simulink model "cable_driven_parallel_robot"  (R2023a)
settings: Solver=ode3  StartTime=0.0  StopTime=100  FixedStep=0.01  RelTol=1e-3
values from neighbouring files (symbols this model uses):
  cable_length = 1.2    [Model_Info.m]
  g = 9.81    [Model_Info.m]
  MP_H = 2    [Model_Info.m]
  MP_init_X = 0    [Model_Info.m]
  MP_init_Y = 0    [Model_Info.m]
  MP_init_Z = cable_length + (MP_H/2)    (= 2.2)    [Model_Info.m]
  MP_Ix = (MP_m/12)*(MP_W^2+MP_H^2)    (= 6.66666666667e-05)    [Model_Info.m]
  MP_Iy = (MP_m/12)*(MP_L^2+MP_H^2)    (= 6.66666666667e-05)    [Model_Info.m]
  MP_Iz = (MP_m/12)*(MP_L^2+MP_W^2)    (= 6.66666666667e-05)    [Model_Info.m]
  MP_L = 2    [Model_Info.m]
  MP_m = 0.0001    [Model_Info.m]
  MP_W = 2    [Model_Info.m]
  MR_init_X_L1 = -(MP_L/2)    (= -1)    [Model_Info.m]
  MR_init_X_L2 = (MP_L/2)    (= 1)    [Model_Info.m]
  MR_init_X_L3 = (MP_L/2)    (= 1)    [Model_Info.m]
  MR_init_X_L4 = -(MP_L/2)    (= -1)    [Model_Info.m]
  MR_init_Y_L1 = -(MP_W/2)    (= -1)    [Model_Info.m]
  MR_init_Y_L2 = -(MP_W/2)    (= -1)    [Model_Info.m]
  MR_init_Y_L3 = (MP_W/2)    (= 1)    [Model_Info.m]
  MR_init_Y_L4 = (MP_W/2)    (= 1)    [Model_Info.m]
  MR_init_Yaw_L1 = pi    (= 3.14159265359)    [Model_Info.m]
  MR_init_Yaw_L2 = 0    [Model_Info.m]
  MR_init_Yaw_L3 = 0    [Model_Info.m]
  MR_init_Yaw_L4 = pi    (= 3.14159265359)    [Model_Info.m]
  MR_Jr = (MR_m/12)*(MR_L^2+MR_W^2)    (= 0.333333333333)    [Model_Info.m]
  MR_m = 0.5    [Model_Info.m]
  MR_r = 2    [Model_Info.m]
  MR_WT = 2    [Model_Info.m]
  QR_Ax = 0.25*0    (= 0)    [Model_Info.m]
  QR_Ay = 0.25*0    (= 0)    [Model_Info.m]
  QR_Az = 0.25*0    (= 0)    [Model_Info.m]
  QR_b = 1.14*1e-7    (= 1.14e-07)    [Model_Info.m]
  QR_Ixx = 4.856*1e-3    (= 0.004856)    [Model_Info.m]
  QR_Iyy = 4.856*1e-3    (= 0.004856)    [Model_Info.m]
  QR_Izz = 8.801*1e-3    (= 0.008801)    [Model_Info.m]
  QR_K = 2.980*1e-6    (= 2.98e-06)    [Model_Info.m]
  QR_l = 0.225    [Model_Info.m]
  QR_m = 0.468    [Model_Info.m]
  QR_x0_U1 = -(MP_L/2)    (= -1)    [Model_Info.m]
  QR_x0_U2 = (MP_L/2)    (= 1)    [Model_Info.m]
  QR_x0_U3 = (MP_L/2)    (= 1)    [Model_Info.m]
  QR_x0_U4 = -(MP_L/2)    (= -1)    [Model_Info.m]
  QR_y0_U1 = -(MP_W/2)    (= -1)    [Model_Info.m]
  QR_y0_U2 = -(MP_W/2)    (= -1)    [Model_Info.m]
  QR_y0_U3 = (MP_W/2)    (= 1)    [Model_Info.m]
  QR_y0_U4 = (MP_W/2)    (= 1)    [Model_Info.m]
  QR_z0_U1 = 2*cable_length+(MP_H)    (= 4.4)    [Model_Info.m]
  QR_z0_U2 = 2*cable_length+(MP_H)    (= 4.4)    [Model_Info.m]
  QR_z0_U3 = 2*cable_length+(MP_H)    (= 4.4)    [Model_Info.m]
  QR_z0_U4 = 2*cable_length+(MP_H)    (= 4.4)    [Model_Info.m]
(part 4 of 12)

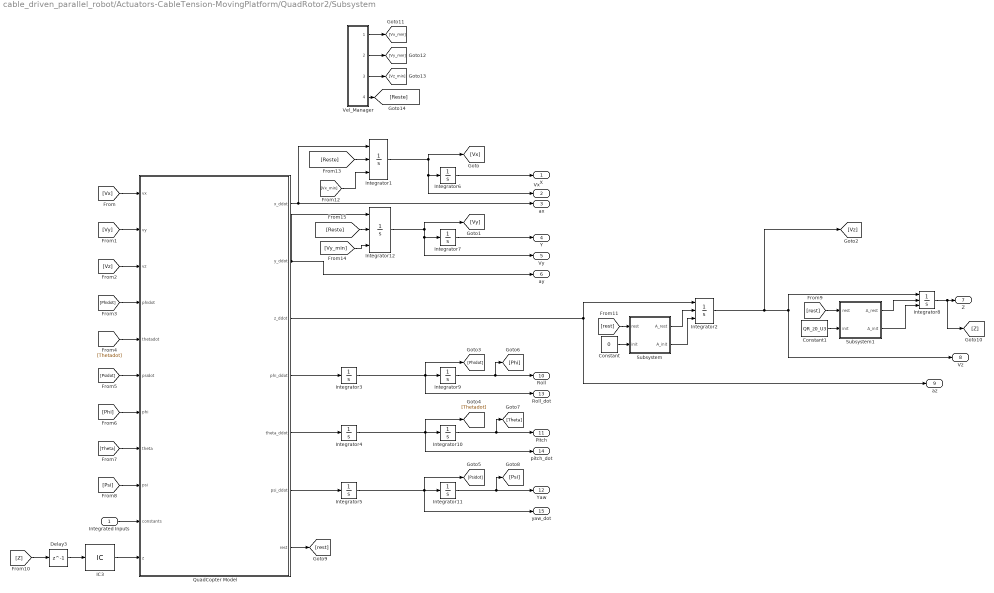
== system cable_driven_parallel_robot/Actuators-CableTension-MovingPlatform/QuadRotor2/Subsystem ==
  Integrated Inputs : Inport
  Constant : Constant  Value=0
  Constant1 : Constant  Value=QR_z0_U3
  Delay3 : Delay  DelayLength=1
  IC3 : InitialCondition  Value=QR_z0_U3
  Integrator1 : Integrator  ExternalReset=rising  InitialConditionSource=external
  Integrator{3..5,9..11} (6 alike) : Integrator
  Integrator12 : Integrator  ExternalReset=rising  InitialConditionSource=external
  Integrator2 : Integrator  ExternalReset=rising  InitialConditionSource=external
  Integrator6 : Integrator  InitialCondition=QR_x0_U3
  Integrator7 : Integrator  InitialCondition=QR_y0_U3
  Integrator8 : Integrator  ExternalReset=rising  InitialConditionSource=external  InitialCondition=QR_z0_U1
  QuadCopter Model : MATLAB Function  TreatAsAtomicUnit=on
  Subsystem : Subsystem
  Subsystem1 : Subsystem
  Vel_Manager : Subsystem
  X : Outport
  Vx : Outport  Port=2
  ax : Outport  Port=3
  Y : Outport  Port=4
  Vy : Outport  Port=5
  ay : Outport  Port=6
  Z : Outport  Port=7
  Vz : Outport  Port=8
  az : Outport  Port=9
  Roll : Outport  Port=10
  Pitch : Outport  Port=11
  Yaw : Outport  Port=12
  Roll_dot : Outport  Port=13
  pitch_dot : Outport  Port=14
  yaw_dot : Outport  Port=15
  wires:
  QuadCopter Model/4(phi_ddot) -> Integrator3/1
  Integrator9/1 -> [Phi], Roll/1
  Integrator4/1 -> pitch_dot/1, [Thetadot], Integrator10/1
  QuadCopter Model/6(psi_ddot) -> Integrator5/1
  Integrator5/1 -> yaw_dot/1, [Psidot], Integrator11/1
  Integrator3/1 -> Roll_dot/1, [Phidot], Integrator9/1
  Integrator1/1 -> [Vx], Vx/1, Integrator6/1
  Integrator10/1 -> [Theta], Pitch/1
  QuadCopter Model/5(theta_ddot) -> Integrator4/1
  QuadCopter Model/2(y_ddot) -> Integrator12/1, ay/1
  QuadCopter Model/1(x_ddot) -> Integrator1/1, ax/1
  Integrator11/1 -> [Psi], Yaw/1
  Integrator6/1 -> X/1
  Integrator7/1 -> Y/1
  Integrator8/1 -> [Z], Z/1
  Integrated Inputs/1 -> QuadCopter Model/10(constants)
  [Vx] -> QuadCopter Model/1(vx)
  [Vy] -> QuadCopter Model/2(vy)
  [Vz] -> QuadCopter Model/3(vz)
  [Phidot] -> QuadCopter Model/4(phidot)
  [Thetadot] -> QuadCopter Model/5(thetadot)
  [Psidot] -> QuadCopter Model/6(psidot)
  [Phi] -> QuadCopter Model/7(phi)
  [Theta] -> QuadCopter Model/8(theta)
  [Psi] -> QuadCopter Model/9(psi)
  Integrator12/1 -> Vy/1, Integrator7/1, [Vy]
  Integrator2/1 -> [Vz], Vz/1, Integrator8/1
  QuadCopter Model/7(rest) -> [rest]
  [Z] -> Delay3/1
  Delay3/1 -> IC3/1
  IC3/1 -> QuadCopter Model/11(z)
  Constant/1 -> Subsystem/2(init)
  [rest] -> Subsystem/1(rest)
  Subsystem/1(A_rest) -> Integrator2/2
  Subsystem/2(A_init) -> Integrator2/3
  [rest] -> Subsystem1/1(rest)
  Subsystem1/1(A_rest) -> Integrator8/2
  Subsystem1/2(A_init) -> Integrator8/3
  Constant1/1 -> Subsystem1/2(init)
  Vel_Manager/4(Reste) -> [Reste]
  Vel_Manager/3(Vz_min) -> [Vz_min]
  Vel_Manager/1(Vx_min) -> [Vx_min]
  Vel_Manager/2(Vy_min) -> [Vy_min]
  [Vx_min] -> Integrator1/3
  [Reste] -> Integrator1/2
  [Vy_min] -> Integrator12/3
  [Reste] -> Integrator12/2
  QuadCopter Model/3(z_ddot) -> az/1, Integrator2/1

== system cable_driven_parallel_robot/Actuators-CableTension-MovingPlatform/QuadRotor3/QuadCopter Inputs ==
  W1 : Inport
  W2 : Inport  Port=2
  W3 : Inport  Port=3
  W4 : Inport  Port=4
  Tx : Inport  Port=5
  Ty : Inport  Port=6
  Tz : Inport  Port=7
  Constant : Constant  Value=QR_Iyy
  Constant1 : Constant  Value=QR_Izz
  Constant10 : Constant  Value=QR_Az
  Constant2 : Constant  Value=g
  Constant3 : Constant  Value=QR_l
  Constant4 : Constant  Value=QR_K
  Constant5 : Constant  Value=QR_b
  Constant6 : Constant  Value=QR_Ax
  Constant7 : Constant  Value=QR_Ay
  Constant8 : Constant  Value=QR_Ixx
  Constant9 : Constant  Value=QR_m
  Mux : Mux  Inputs=18
  Integrated Inputs : Outport
  wires:
  W4/1 -> Mux/15
  W3/1 -> Mux/14
  W2/1 -> Mux/13
  W1/1 -> Mux/12
  Tz/1 -> Mux/18
  Ty/1 -> Mux/17
  Tx/1 -> Mux/16
  Constant2/1 -> Mux/2
  Constant1/1 -> Mux/5
  Constant/1 -> Mux/4
  Constant8/1 -> Mux/3
  Mux/1 -> Integrated Inputs/1
  Constant4/1 -> Mux/7
  Constant7/1 -> Mux/10
  Constant10/1 -> Mux/11
  Constant3/1 -> Mux/6
  Constant9/1 -> Mux/1
  Constant6/1 -> Mux/9
  Constant5/1 -> Mux/8

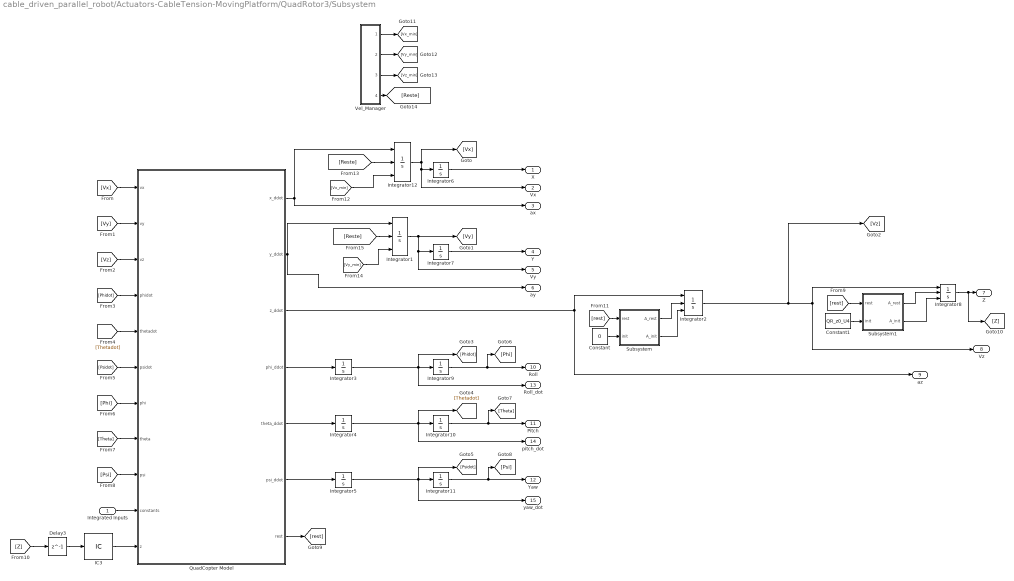
== system cable_driven_parallel_robot/Actuators-CableTension-MovingPlatform/QuadRotor3/Subsystem ==
  Integrated Inputs : Inport
  Constant : Constant  Value=0
  Constant1 : Constant  Value=QR_z0_U4
  Delay3 : Delay  DelayLength=1
  IC3 : InitialCondition  Value=QR_z0_U4
  Integrator1 : Integrator  ExternalReset=rising  InitialConditionSource=external
  Integrator{3..5,9..11} (6 alike) : Integrator
  Integrator12 : Integrator  ExternalReset=rising  InitialConditionSource=external
  Integrator2 : Integrator  ExternalReset=rising  InitialConditionSource=external
  Integrator6 : Integrator  InitialCondition=QR_x0_U4
  Integrator7 : Integrator  InitialCondition=QR_y0_U4
  Integrator8 : Integrator  ExternalReset=rising  InitialConditionSource=external  InitialCondition=QR_z0_U1
  QuadCopter Model : MATLAB Function  TreatAsAtomicUnit=on
  Subsystem : Subsystem
  Subsystem1 : Subsystem
  Vel_Manager : Subsystem
  X : Outport
  Vx : Outport  Port=2
  ax : Outport  Port=3
  Y : Outport  Port=4
  Vy : Outport  Port=5
  ay : Outport  Port=6
  Z : Outport  Port=7
  Vz : Outport  Port=8
  az : Outport  Port=9
  Roll : Outport  Port=10
  Pitch : Outport  Port=11
  Yaw : Outport  Port=12
  Roll_dot : Outport  Port=13
  pitch_dot : Outport  Port=14
  yaw_dot : Outport  Port=15
  wires:
  Constant1/1 -> Subsystem1/2(init)
  Subsystem1/2(A_init) -> Integrator8/3
  Subsystem1/1(A_rest) -> Integrator8/2
  [rest] -> Subsystem1/1(rest)
  Subsystem/2(A_init) -> Integrator2/3
  Subsystem/1(A_rest) -> Integrator2/2
  [rest] -> Subsystem/1(rest)
  Constant/1 -> Subsystem/2(init)
  IC3/1 -> QuadCopter Model/11(z)
  Delay3/1 -> IC3/1
  [Z] -> Delay3/1
  QuadCopter Model/7(rest) -> [rest]
  Integrator2/1 -> [Vz], Integrator8/1, Vz/1
  Integrator1/1 -> Integrator7/1, Vy/1, [Vy]
  [Psi] -> QuadCopter Model/9(psi)
  [Theta] -> QuadCopter Model/8(theta)
  [Phi] -> QuadCopter Model/7(phi)
  [Psidot] -> QuadCopter Model/6(psidot)
  [Thetadot] -> QuadCopter Model/5(thetadot)
  [Phidot] -> QuadCopter Model/4(phidot)
  [Vz] -> QuadCopter Model/3(vz)
  [Vy] -> QuadCopter Model/2(vy)
  [Vx] -> QuadCopter Model/1(vx)
  Integrated Inputs/1 -> QuadCopter Model/10(constants)
  Integrator8/1 -> Z/1, [Z]
  Integrator7/1 -> Y/1
  Integrator6/1 -> X/1
  Integrator11/1 -> Yaw/1, [Psi]
  QuadCopter Model/1(x_ddot) -> Integrator12/1, ax/1
  QuadCopter Model/2(y_ddot) -> Integrator1/1, ay/1
  QuadCopter Model/5(theta_ddot) -> Integrator4/1
  Integrator10/1 -> Pitch/1, [Theta]
  Integrator12/1 -> [Vx], Integrator6/1, Vx/1
  Integrator3/1 -> Integrator9/1, [Phidot], Roll_dot/1
  Integrator5/1 -> Integrator11/1, [Psidot], yaw_dot/1
  QuadCopter Model/6(psi_ddot) -> Integrator5/1
  Integrator4/1 -> Integrator10/1, [Thetadot], pitch_dot/1
  Integrator9/1 -> Roll/1, [Phi]
  QuadCopter Model/4(phi_ddot) -> Integrator3/1
  Vel_Manager/1(Vx_min) -> [Vx_min]
  Vel_Manager/3(Vz_min) -> [Vz_min]
  Vel_Manager/2(Vy_min) -> [Vy_min]
  Vel_Manager/4(Reste) -> [Reste]
  [Vx_min] -> Integrator12/3
  [Reste] -> Integrator12/2
  [Vy_min] -> Integrator1/3
  [Reste] -> Integrator1/2
  QuadCopter Model/3(z_ddot) -> Integrator2/1, az/1

== system cable_driven_parallel_robot/Target Wrench-Jacobian matrix/2 Wheels Diffrential Mobile Robot L1/2 Wheels Diffrential Mobile Robot ==
  TR : Inport
  TL : Inport  Port=2
  mass : Inport  Port=3
  r : Inport  Port=4
  yaw : Inport  Port=5
  x_diff : Inport  Port=6
  y_diff : Inport  Port=7
  z_diff : Inport  Port=8
  x_point : Inport  Port=9
  y_point : Inport  Port=10
  z_point : Inport  Port=11
  2 Wheels Diffrential Mobile Robot : MATLAB Function  TreatAsAtomicUnit=on
  2 Wheels Diffrential Mobile Robot Transformation to Global : MATLAB Function  TreatAsAtomicUnit=on
  Constant : Constant  Value=MR_m
  Constant1 : Constant  Value=cable_length
  Constant2 : Constant  Value=0
  Constant3 : Constant  Value=0
  Delay{1,3,9..10} (4 alike) : Delay  DelayLength=1
  IC1 : InitialCondition  Value=MR_init_Yaw_L1
  IC10 : InitialCondition  Value=MR_init_Y_L1
  IC3 : InitialCondition  Value=0
  IC9 : InitialCondition  Value=MR_init_X_L1
  QR Force Generator : MATLAB Function  TreatAsAtomicUnit=on
  Fx : Outport
  Fy : Outport  Port=2
  Fz : Outport  Port=3
  isTension : Outport  Port=4
  wires:
  TR/1 -> 2 Wheels Diffrential Mobile Robot/1(TR)
  TL/1 -> 2 Wheels Diffrential Mobile Robot/2(TL)
  r/1 -> 2 Wheels Diffrential Mobile Robot/6(r)
  mass/1 -> 2 Wheels Diffrential Mobile Robot/5(mr)
  2 Wheels Diffrential Mobile Robot Transformation to Global/1(Abx) -> [ax]
  2 Wheels Diffrential Mobile Robot Transformation to Global/3(Abz) -> [az]
  2 Wheels Diffrential Mobile Robot Transformation to Global/2(Aby) -> [ay]
  2 Wheels Diffrential Mobile Robot/2(az) -> 2 Wheels Diffrential Mobile Robot Transformation to Global/2(Az)
  2 Wheels Diffrential Mobile Robot/1(ax) -> 2 Wheels Diffrential Mobile Robot Transformation to Global/1(Ax)
  yaw/1 -> Delay1/1
  Delay1/1 -> IC1/1
  IC1/1 -> 2 Wheels Diffrential Mobile Robot Transformation to Global/3(yaw)
  QR Force Generator/3(Fz) -> Fz/1
  Constant/1 -> QR Force Generator/10(mass)
  [ax] -> QR Force Generator/7(ax)
  QR Force Generator/1(Fx) -> Fx/1
  QR Force Generator/2(Fy) -> Fy/1
  [az] -> QR Force Generator/9(az)
  Constant1/1 -> QR Force Generator/11(cable_length)
  [ay] -> QR Force Generator/8(ay)
  Constant3/1 -> 2 Wheels Diffrential Mobile Robot/4(Tz)
  Constant2/1 -> 2 Wheels Diffrential Mobile Robot/3(Tx)
  y_diff/1 -> Delay10/1
  IC10/1 -> QR Force Generator/2(y_diff)
  Delay9/1 -> IC9/1
  x_diff/1 -> Delay9/1
  IC9/1 -> QR Force Generator/1(x_diff)
  Delay10/1 -> IC10/1
  Delay3/1 -> IC3/1
  x_point/1 -> QR Force Generator/4(x_point)
  z_diff/1 -> Delay3/1
  IC3/1 -> QR Force Generator/3(z_diff)
  z_point/1 -> QR Force Generator/6(z_point)
  y_point/1 -> QR Force Generator/5(y_point)
  QR Force Generator/4(isTension) -> isTension/1

== system cable_driven_parallel_robot/Target Wrench-Jacobian matrix/2 Wheels Diffrential Mobile Robot L2/2 Wheels Diffrential Mobile Robot ==
  TR : Inport
  TL : Inport  Port=2
  mass : Inport  Port=3
  r : Inport  Port=4
  yaw : Inport  Port=5
  x_diff : Inport  Port=6
  y_diff : Inport  Port=7
  z_diff : Inport  Port=8
  x_point : Inport  Port=9
  y_point : Inport  Port=10
  z_point : Inport  Port=11
  2 Wheels Diffrential Mobile Robot : MATLAB Function  TreatAsAtomicUnit=on
  2 Wheels Diffrential Mobile Robot Transformation to Global : MATLAB Function  TreatAsAtomicUnit=on
  Constant : Constant  Value=MR_m
  Constant1 : Constant  Value=cable_length
  Constant2 : Constant  Value=0
  Constant3 : Constant  Value=0
  Delay{1,3,9..10} (4 alike) : Delay  DelayLength=1
  IC1 : InitialCondition  Value=MR_init_Yaw_L2
  IC10 : InitialCondition  Value=MR_init_Y_L2
  IC3 : InitialCondition  Value=0
  IC9 : InitialCondition  Value=MR_init_X_L2
  QR Force Generator : MATLAB Function  TreatAsAtomicUnit=on
  Fx : Outport
  Fy : Outport  Port=2
  Fz : Outport  Port=3
  isTension : Outport  Port=4
  wires:
  y_point/1 -> QR Force Generator/5(y_point)
  z_point/1 -> QR Force Generator/6(z_point)
  IC3/1 -> QR Force Generator/3(z_diff)
  z_diff/1 -> Delay3/1
  x_point/1 -> QR Force Generator/4(x_point)
  Delay3/1 -> IC3/1
  Delay10/1 -> IC10/1
  IC9/1 -> QR Force Generator/1(x_diff)
  x_diff/1 -> Delay9/1
  Delay9/1 -> IC9/1
  IC10/1 -> QR Force Generator/2(y_diff)
  y_diff/1 -> Delay10/1
  Constant2/1 -> 2 Wheels Diffrential Mobile Robot/3(Tx)
  Constant3/1 -> 2 Wheels Diffrential Mobile Robot/4(Tz)
  [ay] -> QR Force Generator/8(ay)
  Constant1/1 -> QR Force Generator/11(cable_length)
  [az] -> QR Force Generator/9(az)
  [ax] -> QR Force Generator/7(ax)
  Constant/1 -> QR Force Generator/10(mass)
  IC1/1 -> 2 Wheels Diffrential Mobile Robot Transformation to Global/3(yaw)
  Delay1/1 -> IC1/1
  yaw/1 -> Delay1/1
  2 Wheels Diffrential Mobile Robot/1(ax) -> 2 Wheels Diffrential Mobile Robot Transformation to Global/1(Ax)
  2 Wheels Diffrential Mobile Robot/2(az) -> 2 Wheels Diffrential Mobile Robot Transformation to Global/2(Az)
  2 Wheels Diffrential Mobile Robot Transformation to Global/2(Aby) -> [ay]
  2 Wheels Diffrential Mobile Robot Transformation to Global/3(Abz) -> [az]
  2 Wheels Diffrential Mobile Robot Transformation to Global/1(Abx) -> [ax]
  mass/1 -> 2 Wheels Diffrential Mobile Robot/5(mr)
  r/1 -> 2 Wheels Diffrential Mobile Robot/6(r)
  TL/1 -> 2 Wheels Diffrential Mobile Robot/2(TL)
  TR/1 -> 2 Wheels Diffrential Mobile Robot/1(TR)
  QR Force Generator/2(Fy) -> Fy/1
  QR Force Generator/3(Fz) -> Fz/1
  QR Force Generator/4(isTension) -> isTension/1
  QR Force Generator/1(Fx) -> Fx/1

== system cable_driven_parallel_robot/Target Wrench-Jacobian matrix/2 Wheels Diffrential Mobile Robot L3/2 Wheels Diffrential Mobile Robot ==
  TR : Inport
  TL : Inport  Port=2
  mass : Inport  Port=3
  r : Inport  Port=4
  yaw : Inport  Port=5
  x_diff : Inport  Port=6
  y_diff : Inport  Port=7
  z_diff : Inport  Port=8
  x_point : Inport  Port=9
  y_point : Inport  Port=10
  z_point : Inport  Port=11
  2 Wheels Diffrential Mobile Robot : MATLAB Function  TreatAsAtomicUnit=on
  2 Wheels Diffrential Mobile Robot Transformation to Global : MATLAB Function  TreatAsAtomicUnit=on
  Constant : Constant  Value=MR_m
  Constant1 : Constant  Value=cable_length
  Constant2 : Constant  Value=0
  Constant3 : Constant  Value=0
  Delay{1,3,9..10} (4 alike) : Delay  DelayLength=1
  IC1 : InitialCondition  Value=MR_init_Yaw_L3
  IC10 : InitialCondition  Value=MR_init_Y_L3
  IC3 : InitialCondition  Value=0
  IC9 : InitialCondition  Value=MR_init_X_L3
  QR Force Generator : MATLAB Function  TreatAsAtomicUnit=on
  Fx : Outport
  Fy : Outport  Port=2
  Fz : Outport  Port=3
  isTension : Outport  Port=4
  wires:
  TR/1 -> 2 Wheels Diffrential Mobile Robot/1(TR)
  TL/1 -> 2 Wheels Diffrential Mobile Robot/2(TL)
  r/1 -> 2 Wheels Diffrential Mobile Robot/6(r)
  mass/1 -> 2 Wheels Diffrential Mobile Robot/5(mr)
  2 Wheels Diffrential Mobile Robot Transformation to Global/1(Abx) -> [ax]
  2 Wheels Diffrential Mobile Robot Transformation to Global/3(Abz) -> [az]
  2 Wheels Diffrential Mobile Robot Transformation to Global/2(Aby) -> [ay]
  2 Wheels Diffrential Mobile Robot/2(az) -> 2 Wheels Diffrential Mobile Robot Transformation to Global/2(Az)
  2 Wheels Diffrential Mobile Robot/1(ax) -> 2 Wheels Diffrential Mobile Robot Transformation to Global/1(Ax)
  yaw/1 -> Delay1/1
  Delay1/1 -> IC1/1
  IC1/1 -> 2 Wheels Diffrential Mobile Robot Transformation to Global/3(yaw)
  Constant/1 -> QR Force Generator/10(mass)
  [ax] -> QR Force Generator/7(ax)
  [az] -> QR Force Generator/9(az)
  Constant1/1 -> QR Force Generator/11(cable_length)
  [ay] -> QR Force Generator/8(ay)
  Constant3/1 -> 2 Wheels Diffrential Mobile Robot/4(Tz)
  Constant2/1 -> 2 Wheels Diffrential Mobile Robot/3(Tx)
  y_diff/1 -> Delay10/1
  IC10/1 -> QR Force Generator/2(y_diff)
  Delay9/1 -> IC9/1
  x_diff/1 -> Delay9/1
  IC9/1 -> QR Force Generator/1(x_diff)
  Delay10/1 -> IC10/1
  Delay3/1 -> IC3/1
  x_point/1 -> QR Force Generator/4(x_point)
  z_diff/1 -> Delay3/1
  IC3/1 -> QR Force Generator/3(z_diff)
  z_point/1 -> QR Force Generator/6(z_point)
  y_point/1 -> QR Force Generator/5(y_point)
  QR Force Generator/2(Fy) -> Fy/1
  QR Force Generator/3(Fz) -> Fz/1
  QR Force Generator/4(isTension) -> isTension/1
  QR Force Generator/1(Fx) -> Fx/1

== system cable_driven_parallel_robot/Target Wrench-Jacobian matrix/2 Wheels Diffrential Mobile Robot L4/2 Wheels Diffrential Mobile Robot ==
  TR : Inport
  TL : Inport  Port=2
  mass : Inport  Port=3
  r : Inport  Port=4
  yaw : Inport  Port=5
  x_diff : Inport  Port=6
  y_diff : Inport  Port=7
  z_diff : Inport  Port=8
  x_point : Inport  Port=9
  y_point : Inport  Port=10
  z_point : Inport  Port=11
  2 Wheels Diffrential Mobile Robot : MATLAB Function  TreatAsAtomicUnit=on
  2 Wheels Diffrential Mobile Robot Transformation to Global : MATLAB Function  TreatAsAtomicUnit=on
  Constant : Constant  Value=MR_m
  Constant1 : Constant  Value=cable_length
  Constant2 : Constant  Value=0
  Constant3 : Constant  Value=0
  Delay{1,3,9..10} (4 alike) : Delay  DelayLength=1
  IC1 : InitialCondition  Value=MR_init_Yaw_L4
  IC10 : InitialCondition  Value=MR_init_Y_L4
  IC3 : InitialCondition  Value=0
  IC9 : InitialCondition  Value=MR_init_X_L4
  QR Force Generator : MATLAB Function  TreatAsAtomicUnit=on
  Fx : Outport
  Fy : Outport  Port=2
  Fz : Outport  Port=3
  isTension : Outport  Port=4
  wires:
  y_point/1 -> QR Force Generator/5(y_point)
  z_point/1 -> QR Force Generator/6(z_point)
  IC3/1 -> QR Force Generator/3(z_diff)
  z_diff/1 -> Delay3/1
  x_point/1 -> QR Force Generator/4(x_point)
  Delay3/1 -> IC3/1
  Delay10/1 -> IC10/1
  IC9/1 -> QR Force Generator/1(x_diff)
  x_diff/1 -> Delay9/1
  Delay9/1 -> IC9/1
  IC10/1 -> QR Force Generator/2(y_diff)
  y_diff/1 -> Delay10/1
  Constant2/1 -> 2 Wheels Diffrential Mobile Robot/3(Tx)
  Constant3/1 -> 2 Wheels Diffrential Mobile Robot/4(Tz)
  [ay] -> QR Force Generator/8(ay)
  Constant1/1 -> QR Force Generator/11(cable_length)
  [az] -> QR Force Generator/9(az)
  [ax] -> QR Force Generator/7(ax)
  Constant/1 -> QR Force Generator/10(mass)
  IC1/1 -> 2 Wheels Diffrential Mobile Robot Transformation to Global/3(yaw)
  Delay1/1 -> IC1/1
  yaw/1 -> Delay1/1
  2 Wheels Diffrential Mobile Robot/1(ax) -> 2 Wheels Diffrential Mobile Robot Transformation to Global/1(Ax)
  2 Wheels Diffrential Mobile Robot/2(az) -> 2 Wheels Diffrential Mobile Robot Transformation to Global/2(Az)
  2 Wheels Diffrential Mobile Robot Transformation to Global/2(Aby) -> [ay]
  2 Wheels Diffrential Mobile Robot Transformation to Global/3(Abz) -> [az]
  2 Wheels Diffrential Mobile Robot Transformation to Global/1(Abx) -> [ax]
  mass/1 -> 2 Wheels Diffrential Mobile Robot/5(mr)
  r/1 -> 2 Wheels Diffrential Mobile Robot/6(r)
  TL/1 -> 2 Wheels Diffrential Mobile Robot/2(TL)
  TR/1 -> 2 Wheels Diffrential Mobile Robot/1(TR)
  QR Force Generator/2(Fy) -> Fy/1
  QR Force Generator/3(Fz) -> Fz/1
  QR Force Generator/4(isTension) -> isTension/1
  QR Force Generator/1(Fx) -> Fx/1

== system cable_driven_parallel_robot/Target Wrench-Jacobian matrix/Moving Platform/Moving Platform ==
  mass : Inport
  QR Force Generator : MATLAB Function  TreatAsAtomicUnit=on
  Fx : Outport
  Fy : Outport  Port=2
  Fz : Outport  Port=3
  wires:
  QR Force Generator/2(Fy) -> Fy/1
  QR Force Generator/3(Fz) -> Fz/1
  QR Force Generator/1(Fx) -> Fx/1
  mass/1 -> QR Force Generator/1(mass)

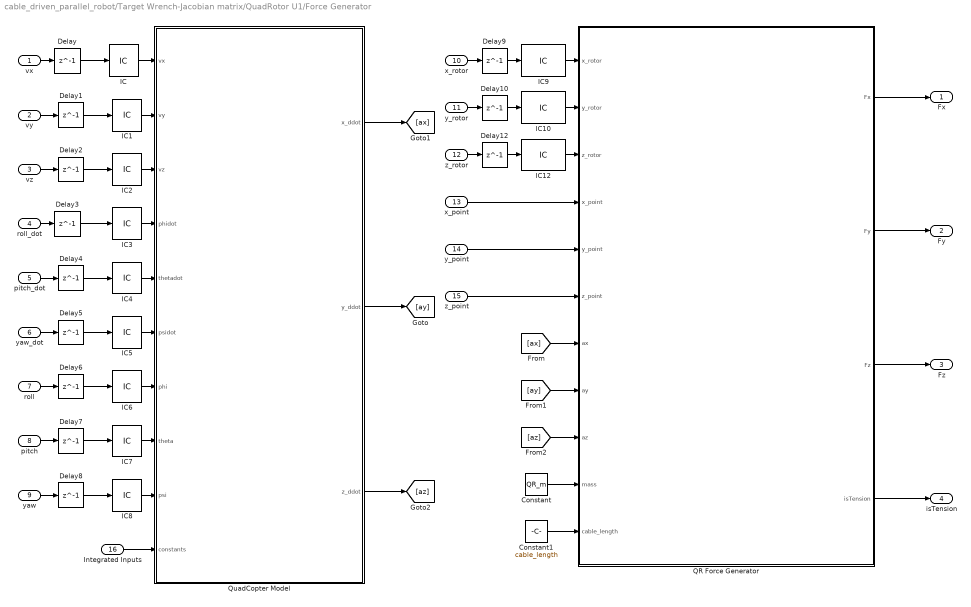
== system cable_driven_parallel_robot/Target Wrench-Jacobian matrix/QuadRotor U1/Force Generator ==
  vx : Inport
  vy : Inport  Port=2
  vz : Inport  Port=3
  roll_dot : Inport  Port=4
  pitch_dot : Inport  Port=5
  yaw_dot : Inport  Port=6
  roll : Inport  Port=7
  pitch : Inport  Port=8
  yaw : Inport  Port=9
  x_rotor : Inport  Port=10
  y_rotor : Inport  Port=11
  z_rotor : Inport  Port=12
  x_point : Inport  Port=13
  y_point : Inport  Port=14
  z_point : Inport  Port=15
  Integrated Inputs : Inport  Port=16
  Constant : Constant  Value=QR_m
  Constant1 : Constant  Value=cable_length
  Delay{,1..10,12} (12 alike) : Delay  DelayLength=1
  IC{,1..8} (9 alike) : InitialCondition  Value=0
  IC10 : InitialCondition  Value=QR_y0_U1
  IC12 : InitialCondition  Value=QR_z0_U1
  IC9 : InitialCondition  Value=QR_x0_U1
  QR Force Generator : MATLAB Function  TreatAsAtomicUnit=on
  QuadCopter Model : MATLAB Function  TreatAsAtomicUnit=on
  Fx : Outport
  Fy : Outport  Port=2
  Fz : Outport  Port=3
  isTension : Outport  Port=4
  wires:
  QuadCopter Model/2(y_ddot) -> [ay]
  QuadCopter Model/1(x_ddot) -> [ax]
  Integrated Inputs/1 -> QuadCopter Model/10(constants)
  QuadCopter Model/3(z_ddot) -> [az]
  [ax] -> QR Force Generator/7(ax)
  [ay] -> QR Force Generator/8(ay)
  [az] -> QR Force Generator/9(az)
  Constant/1 -> QR Force Generator/10(mass)
  Constant1/1 -> QR Force Generator/11(cable_length)
  QR Force Generator/1(Fx) -> Fx/1
  QR Force Generator/2(Fy) -> Fy/1
  QR Force Generator/3(Fz) -> Fz/1
  vx/1 -> Delay/1
  Delay/1 -> IC/1
  IC/1 -> QuadCopter Model/1(vx)
  vy/1 -> Delay1/1
  Delay1/1 -> IC1/1
  IC1/1 -> QuadCopter Model/2(vy)
  IC2/1 -> QuadCopter Model/3(vz)
  vz/1 -> Delay2/1
  Delay2/1 -> IC2/1
  roll_dot/1 -> Delay3/1
  IC4/1 -> QuadCopter Model/5(thetadot)
  Delay5/1 -> IC5/1
  Delay3/1 -> IC3/1
  IC3/1 -> QuadCopter Model/4(phidot)
  pitch_dot/1 -> Delay4/1
  Delay4/1 -> IC4/1
  IC5/1 -> QuadCopter Model/6(psidot)
  yaw_dot/1 -> Delay5/1
  roll/1 -> Delay6/1
  IC7/1 -> QuadCopter Model/8(theta)
  Delay8/1 -> IC8/1
  Delay6/1 -> IC6/1
  IC6/1 -> QuadCopter Model/7(phi)
  pitch/1 -> Delay7/1
  Delay7/1 -> IC7/1
  IC8/1 -> QuadCopter Model/9(psi)
  yaw/1 -> Delay8/1
  IC9/1 -> QR Force Generator/1(x_rotor)
  x_rotor/1 -> Delay9/1
  Delay9/1 -> IC9/1
  Delay10/1 -> IC10/1
  y_rotor/1 -> Delay10/1
  IC10/1 -> QR Force Generator/2(y_rotor)
  x_point/1 -> QR Force Generator/4(x_point)
  Delay12/1 -> IC12/1
  z_rotor/1 -> Delay12/1
  IC12/1 -> QR Force Generator/3(z_rotor)
  z_point/1 -> QR Force Generator/6(z_point)
  y_point/1 -> QR Force Generator/5(y_point)
  QR Force Generator/4(isTension) -> isTension/1

== system cable_driven_parallel_robot/Target Wrench-Jacobian matrix/QuadRotor U1/QuadCopter Inputs ==
  W1 : Inport
  W2 : Inport  Port=2
  W3 : Inport  Port=3
  W4 : Inport  Port=4
  Tx : Inport  Port=5
  Ty : Inport  Port=6
  Tz : Inport  Port=7
  Constant : Constant  Value=QR_Iyy
  Constant1 : Constant  Value=QR_Izz
  Constant10 : Constant  Value=QR_Az
  Constant2 : Constant  Value=g
  Constant3 : Constant  Value=QR_l
  Constant4 : Constant  Value=QR_K
  Constant5 : Constant  Value=QR_b
  Constant6 : Constant  Value=QR_Ax
  Constant7 : Constant  Value=QR_Ay
  Constant8 : Constant  Value=QR_Ixx
  Constant9 : Constant  Value=QR_m
  Mux : Mux  Inputs=18
  Integrated Inputs : Outport
  wires:
  Constant5/1 -> Mux/8
  Constant6/1 -> Mux/9
  Constant9/1 -> Mux/1
  Constant3/1 -> Mux/6
  Constant10/1 -> Mux/11
  Constant7/1 -> Mux/10
  Constant4/1 -> Mux/7
  Mux/1 -> Integrated Inputs/1
  Constant8/1 -> Mux/3
  Constant/1 -> Mux/4
  Constant1/1 -> Mux/5
  Constant2/1 -> Mux/2
  Tx/1 -> Mux/16
  Ty/1 -> Mux/17
  Tz/1 -> Mux/18
  W1/1 -> Mux/12
  W2/1 -> Mux/13
  W3/1 -> Mux/14
  W4/1 -> Mux/15

== system cable_driven_parallel_robot/Target Wrench-Jacobian matrix/QuadRotor U2/Force Generator ==
  vx : Inport
  vy : Inport  Port=2
  vz : Inport  Port=3
  roll_dot : Inport  Port=4
  pitch_dot : Inport  Port=5
  yaw_dot : Inport  Port=6
  roll : Inport  Port=7
  pitch : Inport  Port=8
  yaw : Inport  Port=9
  x_rotor : Inport  Port=10
  y_rotor : Inport  Port=11
  z_rotor : Inport  Port=12
  x_point : Inport  Port=13
  y_point : Inport  Port=14
  z_point : Inport  Port=15
  Integrated Inputs : Inport  Port=16
  Constant : Constant  Value=QR_m
  Constant1 : Constant  Value=cable_length
  Delay{,1..10,12} (12 alike) : Delay  DelayLength=1
  IC{,1..8} (9 alike) : InitialCondition  Value=0
  IC10 : InitialCondition  Value=QR_y0_U2
  IC12 : InitialCondition  Value=QR_z0_U2
  IC9 : InitialCondition  Value=QR_x0_U2
  QR Force Generator : MATLAB Function  TreatAsAtomicUnit=on
  QuadCopter Model : MATLAB Function  TreatAsAtomicUnit=on
  Fx : Outport
  Fy : Outport  Port=2
  Fz : Outport  Port=3
  isTension : Outport  Port=4
  wires:
  QuadCopter Model/2(y_ddot) -> [ay]
  QuadCopter Model/1(x_ddot) -> [ax]
  Integrated Inputs/1 -> QuadCopter Model/10(constants)
  QuadCopter Model/3(z_ddot) -> [az]
  [ax] -> QR Force Generator/7(ax)
  [ay] -> QR Force Generator/8(ay)
  [az] -> QR Force Generator/9(az)
  Constant/1 -> QR Force Generator/10(mass)
  Constant1/1 -> QR Force Generator/11(cable_length)
  vx/1 -> Delay/1
  Delay/1 -> IC/1
  IC/1 -> QuadCopter Model/1(vx)
  vy/1 -> Delay1/1
  Delay1/1 -> IC1/1
  IC1/1 -> QuadCopter Model/2(vy)
  IC2/1 -> QuadCopter Model/3(vz)
  vz/1 -> Delay2/1
  Delay2/1 -> IC2/1
  roll_dot/1 -> Delay3/1
  IC4/1 -> QuadCopter Model/5(thetadot)
  Delay5/1 -> IC5/1
  Delay3/1 -> IC3/1
  IC3/1 -> QuadCopter Model/4(phidot)
  pitch_dot/1 -> Delay4/1
  Delay4/1 -> IC4/1
  IC5/1 -> QuadCopter Model/6(psidot)
  yaw_dot/1 -> Delay5/1
  roll/1 -> Delay6/1
  IC7/1 -> QuadCopter Model/8(theta)
  Delay8/1 -> IC8/1
  Delay6/1 -> IC6/1
  IC6/1 -> QuadCopter Model/7(phi)
  pitch/1 -> Delay7/1
  Delay7/1 -> IC7/1
  IC8/1 -> QuadCopter Model/9(psi)
  yaw/1 -> Delay8/1
  IC9/1 -> QR Force Generator/1(x_rotor)
  x_rotor/1 -> Delay9/1
  Delay9/1 -> IC9/1
  Delay10/1 -> IC10/1
  y_rotor/1 -> Delay10/1
  IC10/1 -> QR Force Generator/2(y_rotor)
  x_point/1 -> QR Force Generator/4(x_point)
  Delay12/1 -> IC12/1
  z_rotor/1 -> Delay12/1
  IC12/1 -> QR Force Generator/3(z_rotor)
  z_point/1 -> QR Force Generator/6(z_point)
  y_point/1 -> QR Force Generator/5(y_point)
  QR Force Generator/4(isTension) -> isTension/1
  QR Force Generator/2(Fy) -> Fy/1
  QR Force Generator/3(Fz) -> Fz/1
  QR Force Generator/1(Fx) -> Fx/1

== system cable_driven_parallel_robot/Target Wrench-Jacobian matrix/QuadRotor U2/QuadCopter Inputs ==
  W1 : Inport
  W2 : Inport  Port=2
  W3 : Inport  Port=3
  W4 : Inport  Port=4
  Tx : Inport  Port=5
  Ty : Inport  Port=6
  Tz : Inport  Port=7
  Constant : Constant  Value=QR_Iyy
  Constant1 : Constant  Value=QR_Izz
  Constant10 : Constant  Value=QR_Az
  Constant2 : Constant  Value=g
  Constant3 : Constant  Value=QR_l
  Constant4 : Constant  Value=QR_K
  Constant5 : Constant  Value=QR_b
  Constant6 : Constant  Value=QR_Ax
  Constant7 : Constant  Value=QR_Ay
  Constant8 : Constant  Value=QR_Ixx
  Constant9 : Constant  Value=QR_m
  Mux : Mux  Inputs=18
  Integrated Inputs : Outport
  wires:
  Constant5/1 -> Mux/8
  Constant6/1 -> Mux/9
  Constant9/1 -> Mux/1
  Constant3/1 -> Mux/6
  Constant10/1 -> Mux/11
  Constant7/1 -> Mux/10
  Constant4/1 -> Mux/7
  Mux/1 -> Integrated Inputs/1
  Constant8/1 -> Mux/3
  Constant/1 -> Mux/4
  Constant1/1 -> Mux/5
  Constant2/1 -> Mux/2
  Tx/1 -> Mux/16
  Ty/1 -> Mux/17
  Tz/1 -> Mux/18
  W1/1 -> Mux/12
  W2/1 -> Mux/13
  W3/1 -> Mux/14
  W4/1 -> Mux/15

== system cable_driven_parallel_robot/Target Wrench-Jacobian matrix/QuadRotor U3/Force Generator ==
  vx : Inport
  vy : Inport  Port=2
  vz : Inport  Port=3
  roll_dot : Inport  Port=4
  pitch_dot : Inport  Port=5
  yaw_dot : Inport  Port=6
  roll : Inport  Port=7
  pitch : Inport  Port=8
  yaw : Inport  Port=9
  x_rotor : Inport  Port=10
  y_rotor : Inport  Port=11
  z_rotor : Inport  Port=12
  x_point : Inport  Port=13
  y_point : Inport  Port=14
  z_point : Inport  Port=15
  Integrated Inputs : Inport  Port=16
  Constant : Constant  Value=QR_m
  Constant1 : Constant  Value=cable_length
  Delay{,1..10,12} (12 alike) : Delay  DelayLength=1
  IC{,1..8} (9 alike) : InitialCondition  Value=0
  IC10 : InitialCondition  Value=QR_y0_U3
  IC12 : InitialCondition  Value=QR_z0_U3
  IC9 : InitialCondition  Value=QR_x0_U3
  QR Force Generator : MATLAB Function  TreatAsAtomicUnit=on
  QuadCopter Model : MATLAB Function  TreatAsAtomicUnit=on
  Fx : Outport
  Fy : Outport  Port=2
  Fz : Outport  Port=3
  isTension : Outport  Port=4
  wires:
  y_point/1 -> QR Force Generator/5(y_point)
  z_point/1 -> QR Force Generator/6(z_point)
  IC12/1 -> QR Force Generator/3(z_rotor)
  z_rotor/1 -> Delay12/1
  Delay12/1 -> IC12/1
  x_point/1 -> QR Force Generator/4(x_point)
  IC10/1 -> QR Force Generator/2(y_rotor)
  y_rotor/1 -> Delay10/1
  Delay10/1 -> IC10/1
  Delay9/1 -> IC9/1
  x_rotor/1 -> Delay9/1
  IC9/1 -> QR Force Generator/1(x_rotor)
  yaw/1 -> Delay8/1
  IC8/1 -> QuadCopter Model/9(psi)
  Delay7/1 -> IC7/1
  pitch/1 -> Delay7/1
  IC6/1 -> QuadCopter Model/7(phi)
  Delay6/1 -> IC6/1
  Delay8/1 -> IC8/1
  IC7/1 -> QuadCopter Model/8(theta)
  roll/1 -> Delay6/1
  yaw_dot/1 -> Delay5/1
  IC5/1 -> QuadCopter Model/6(psidot)
  Delay4/1 -> IC4/1
  pitch_dot/1 -> Delay4/1
  IC3/1 -> QuadCopter Model/4(phidot)
  Delay3/1 -> IC3/1
  Delay5/1 -> IC5/1
  IC4/1 -> QuadCopter Model/5(thetadot)
  roll_dot/1 -> Delay3/1
  Delay2/1 -> IC2/1
  vz/1 -> Delay2/1
  IC2/1 -> QuadCopter Model/3(vz)
  IC1/1 -> QuadCopter Model/2(vy)
  Delay1/1 -> IC1/1
  vy/1 -> Delay1/1
  IC/1 -> QuadCopter Model/1(vx)
  Delay/1 -> IC/1
  vx/1 -> Delay/1
  Constant1/1 -> QR Force Generator/11(cable_length)
  Constant/1 -> QR Force Generator/10(mass)
  [az] -> QR Force Generator/9(az)
  [ay] -> QR Force Generator/8(ay)
  [ax] -> QR Force Generator/7(ax)
  QuadCopter Model/3(z_ddot) -> [az]
  Integrated Inputs/1 -> QuadCopter Model/10(constants)
  QuadCopter Model/1(x_ddot) -> [ax]
  QuadCopter Model/2(y_ddot) -> [ay]
  QR Force Generator/4(isTension) -> isTension/1
  QR Force Generator/2(Fy) -> Fy/1
  QR Force Generator/3(Fz) -> Fz/1
  QR Force Generator/1(Fx) -> Fx/1

== system cable_driven_parallel_robot/Target Wrench-Jacobian matrix/QuadRotor U3/QuadCopter Inputs ==
  W1 : Inport
  W2 : Inport  Port=2
  W3 : Inport  Port=3
  W4 : Inport  Port=4
  Tx : Inport  Port=5
  Ty : Inport  Port=6
  Tz : Inport  Port=7
  Constant : Constant  Value=QR_Iyy
  Constant1 : Constant  Value=QR_Izz
  Constant10 : Constant  Value=QR_Az
  Constant2 : Constant  Value=g
  Constant3 : Constant  Value=QR_l
  Constant4 : Constant  Value=QR_K
  Constant5 : Constant  Value=QR_b
  Constant6 : Constant  Value=QR_Ax
  Constant7 : Constant  Value=QR_Ay
  Constant8 : Constant  Value=QR_Ixx
  Constant9 : Constant  Value=QR_m
  Mux : Mux  Inputs=18
  Integrated Inputs : Outport
  wires:
  W4/1 -> Mux/15
  W3/1 -> Mux/14
  W2/1 -> Mux/13
  W1/1 -> Mux/12
  Tz/1 -> Mux/18
  Ty/1 -> Mux/17
  Tx/1 -> Mux/16
  Constant2/1 -> Mux/2
  Constant1/1 -> Mux/5
  Constant/1 -> Mux/4
  Constant8/1 -> Mux/3
  Mux/1 -> Integrated Inputs/1
  Constant4/1 -> Mux/7
  Constant7/1 -> Mux/10
  Constant10/1 -> Mux/11
  Constant3/1 -> Mux/6
  Constant9/1 -> Mux/1
  Constant6/1 -> Mux/9
  Constant5/1 -> Mux/8

== system cable_driven_parallel_robot/Target Wrench-Jacobian matrix/QuadRotor U4/Force Generator ==
  vx : Inport
  vy : Inport  Port=2
  vz : Inport  Port=3
  roll_dot : Inport  Port=4
  pitch_dot : Inport  Port=5
  yaw_dot : Inport  Port=6
  roll : Inport  Port=7
  pitch : Inport  Port=8
  yaw : Inport  Port=9
  x_rotor : Inport  Port=10
  y_rotor : Inport  Port=11
  z_rotor : Inport  Port=12
  x_point : Inport  Port=13
  y_point : Inport  Port=14
  z_point : Inport  Port=15
  Integrated Inputs : Inport  Port=16
  Constant : Constant  Value=QR_m
  Constant1 : Constant  Value=cable_length
  Delay{,1..10,12} (12 alike) : Delay  DelayLength=1
  IC{,1..8} (9 alike) : InitialCondition  Value=0
  IC10 : InitialCondition  Value=QR_y0_U4
  IC12 : InitialCondition  Value=QR_z0_U4
  IC9 : InitialCondition  Value=QR_x0_U4
  QR Force Generator : MATLAB Function  TreatAsAtomicUnit=on
  QuadCopter Model : MATLAB Function  TreatAsAtomicUnit=on
  Fx : Outport
  Fy : Outport  Port=2
  Fz : Outport  Port=3
  isTension : Outport  Port=4
  wires:
  QuadCopter Model/2(y_ddot) -> [ay]
  QuadCopter Model/1(x_ddot) -> [ax]
  Integrated Inputs/1 -> QuadCopter Model/10(constants)
  QuadCopter Model/3(z_ddot) -> [az]
  [ax] -> QR Force Generator/7(ax)
  [ay] -> QR Force Generator/8(ay)
  [az] -> QR Force Generator/9(az)
  Constant/1 -> QR Force Generator/10(mass)
  Constant1/1 -> QR Force Generator/11(cable_length)
  vx/1 -> Delay/1
  Delay/1 -> IC/1
  IC/1 -> QuadCopter Model/1(vx)
  vy/1 -> Delay1/1
  Delay1/1 -> IC1/1
  IC1/1 -> QuadCopter Model/2(vy)
  IC2/1 -> QuadCopter Model/3(vz)
  vz/1 -> Delay2/1
  Delay2/1 -> IC2/1
  roll_dot/1 -> Delay3/1
  IC4/1 -> QuadCopter Model/5(thetadot)
  Delay5/1 -> IC5/1
  Delay3/1 -> IC3/1
  IC3/1 -> QuadCopter Model/4(phidot)
  pitch_dot/1 -> Delay4/1
  Delay4/1 -> IC4/1
  IC5/1 -> QuadCopter Model/6(psidot)
  yaw_dot/1 -> Delay5/1
  roll/1 -> Delay6/1
  IC7/1 -> QuadCopter Model/8(theta)
  Delay8/1 -> IC8/1
  Delay6/1 -> IC6/1
  IC6/1 -> QuadCopter Model/7(phi)
  pitch/1 -> Delay7/1
  Delay7/1 -> IC7/1
  IC8/1 -> QuadCopter Model/9(psi)
  yaw/1 -> Delay8/1
  IC9/1 -> QR Force Generator/1(x_rotor)
  x_rotor/1 -> Delay9/1
  Delay9/1 -> IC9/1
  Delay10/1 -> IC10/1
  y_rotor/1 -> Delay10/1
  IC10/1 -> QR Force Generator/2(y_rotor)
  x_point/1 -> QR Force Generator/4(x_point)
  Delay12/1 -> IC12/1
  z_rotor/1 -> Delay12/1
  IC12/1 -> QR Force Generator/3(z_rotor)
  z_point/1 -> QR Force Generator/6(z_point)
  y_point/1 -> QR Force Generator/5(y_point)
  QR Force Generator/4(isTension) -> isTension/1
  QR Force Generator/2(Fy) -> Fy/1
  QR Force Generator/3(Fz) -> Fz/1
  QR Force Generator/1(Fx) -> Fx/1

== system cable_driven_parallel_robot/Target Wrench-Jacobian matrix/QuadRotor U4/QuadCopter Inputs ==
  W1 : Inport
  W2 : Inport  Port=2
  W3 : Inport  Port=3
  W4 : Inport  Port=4
  Tx : Inport  Port=5
  Ty : Inport  Port=6
  Tz : Inport  Port=7
  Constant : Constant  Value=QR_Iyy
  Constant1 : Constant  Value=QR_Izz
  Constant10 : Constant  Value=QR_Az
  Constant2 : Constant  Value=g
  Constant3 : Constant  Value=QR_l
  Constant4 : Constant  Value=QR_K
  Constant5 : Constant  Value=QR_b
  Constant6 : Constant  Value=QR_Ax
  Constant7 : Constant  Value=QR_Ay
  Constant8 : Constant  Value=QR_Ixx
  Constant9 : Constant  Value=QR_m
  Mux : Mux  Inputs=18
  Integrated Inputs : Outport
  wires:
  Constant5/1 -> Mux/8
  Constant6/1 -> Mux/9
  Constant9/1 -> Mux/1
  Constant3/1 -> Mux/6
  Constant10/1 -> Mux/11
  Constant7/1 -> Mux/10
  Constant4/1 -> Mux/7
  Mux/1 -> Integrated Inputs/1
  Constant8/1 -> Mux/3
  Constant/1 -> Mux/4
  Constant1/1 -> Mux/5
  Constant2/1 -> Mux/2
  Tx/1 -> Mux/16
  Ty/1 -> Mux/17
  Tz/1 -> Mux/18
  W1/1 -> Mux/12
  W2/1 -> Mux/13
  W3/1 -> Mux/14
  W4/1 -> Mux/15

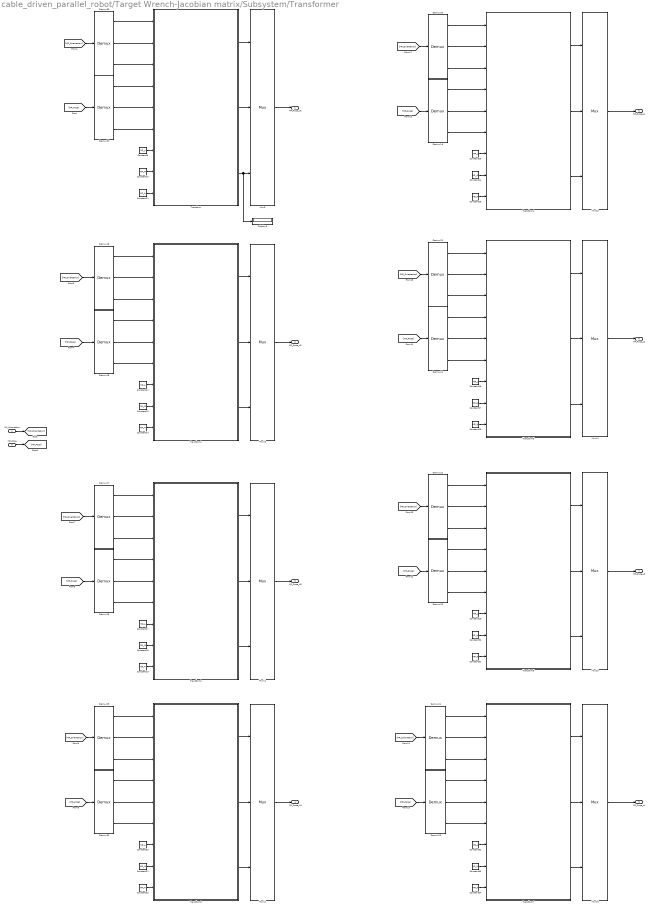
== system cable_driven_parallel_robot/Target Wrench-Jacobian matrix/Subsystem/Transformer ==
  MP_Orientation : Inport
  MP_Pose : Inport  Port=2
  Constant{10,13,18,21,24,27,30,33} (8 alike) : Constant  Value=MP_W
  Constant{11,14,19,22,25,28,31,34} (8 alike) : Constant  Value=MP_H
  Constant{9,12,17,20,23,26,29,32} (8 alike) : Constant  Value=MP_L
  Demux{18..33} (16 alike) : Demux  Outputs=3
  Display3 : Display
  Mux{9..16} (8 alike) : Mux  Inputs=3
  Transform : MATLAB Function  TreatAsAtomicUnit=on
  Transform1 : MATLAB Function  TreatAsAtomicUnit=on
  Transform2 : MATLAB Function  TreatAsAtomicUnit=on
  Transform3 : MATLAB Function  TreatAsAtomicUnit=on
  Transform4 : MATLAB Function  TreatAsAtomicUnit=on
  Transform5 : MATLAB Function  TreatAsAtomicUnit=on
  Transform6 : MATLAB Function  TreatAsAtomicUnit=on
  Transform7 : MATLAB Function  TreatAsAtomicUnit=on
  MP_Pose_U1 : Outport
  MP_Pose_U2 : Outport  Port=2
  MP_Pose_U3 : Outport  Port=3
  MP_Pose_U4 : Outport  Port=4
  MP_Pose_L1 : Outport  Port=5
  MP_Pose_L2 : Outport  Port=6
  MP_Pose_L3 : Outport  Port=7
  MP_Pose_L4 : Outport  Port=8
  wires:
  Constant13/1 -> Transform1/8(W)
  Constant12/1 -> Transform1/7(L)
  Transform1/1(MP_U2_X) -> Mux10/1
  Mux11/1 -> MP_Pose_U3/1
  Transform1/2(MP_U2_Y) -> Mux10/2
  Constant14/1 -> Transform1/9(H)
  Transform4/1(MP_L1_X) -> Mux13/1
  Constant29/1 -> Transform6/7(L)
  Mux14/1 -> MP_Pose_L2/1
  Constant34/1 -> Transform7/9(H)
  Transform2/1(MP_U3_X) -> Mux11/1
  Constant18/1 -> Transform2/8(W)
  Mux9/1 -> MP_Pose_U1/1
  Transform7/2(MP_L4_Y) -> Mux16/2
  Transform2/2(MP_U3_Y) -> Mux11/2
  Transform/2(MP_U1_Y) -> Mux9/2
  Constant23/1 -> Transform4/7(L)
  Constant32/1 -> Transform7/7(L)
  Constant17/1 -> Transform2/7(L)
  Constant9/1 -> Transform/7(L)
  Transform7/1(MP_L4_X) -> Mux16/1
  Transform/1(MP_U1_X) -> Mux9/1
  Constant10/1 -> Transform/8(W)
  Constant11/1 -> Transform/9(H)
  Transform6/2(MP_L3_Y) -> Mux15/2
  Constant19/1 -> Transform2/9(H)
  Mux10/1 -> MP_Pose_U2/1
  Transform5/2(MP_L2_Y) -> Mux14/2
  Constant33/1 -> Transform7/8(W)
  Mux16/1 -> MP_Pose_L4/1
  Mux15/1 -> MP_Pose_L3/1
  Constant26/1 -> Transform5/7(L)
  Mux13/1 -> MP_Pose_L1/1
  Constant25/1 -> Transform4/9(H)
  Transform4/2(MP_L1_Y) -> Mux13/2
  Constant31/1 -> Transform6/9(H)
  Transform6/1(MP_L3_X) -> Mux15/1
  Mux12/1 -> MP_Pose_U4/1
  Constant22/1 -> Transform3/9(H)
  Constant24/1 -> Transform4/8(W)
  Transform3/2(MP_U4_Y) -> Mux12/2
  Constant28/1 -> Transform5/9(H)
  Transform5/1(MP_L2_X) -> Mux14/1
  Constant27/1 -> Transform5/8(W)
  Constant20/1 -> Transform3/7(L)
  Constant21/1 -> Transform3/8(W)
  [MP_Pose] -> Demux28/1
  Constant30/1 -> Transform6/8(W)
  Transform3/1(MP_U4_X) -> Mux12/1
  [MP_Orientation] -> Demux18/1
  [MP_Orientation] -> Demux27/1
  [MP_Pose] -> Demux26/1
  MP_Orientation/1 -> [MP_Orientation]
  MP_Pose/1 -> [MP_Pose]
  [MP_Orientation] -> Demux30/1
  [MP_Pose] -> Demux31/1
  [MP_Orientation] -> Demux29/1
  [MP_Pose] -> Demux32/1
  [MP_Orientation] -> Demux24/1
  [MP_Pose] -> Demux25/1
  [MP_Orientation] -> Demux22/1
  [MP_Pose] -> Demux23/1
  [MP_Orientation] -> Demux20/1
  [MP_Pose] -> Demux21/1
  [MP_Orientation] -> Demux33/1
  [MP_Pose] -> Demux19/1
  Demux30/3 -> Transform/3(yaw)
  Demux30/1 -> Transform/1(roll)
  Demux30/2 -> Transform/2(pitch)
  Demux31/2 -> Transform/5(MP_Y)
  Demux31/1 -> Transform/4(MP_X)
  Demux18/3 -> Transform1/3(yaw)
  Demux26/3 -> Transform1/6(MP_Z)
  Demux26/2 -> Transform1/5(MP_Y)
  Demux26/1 -> Transform1/4(MP_X)
  Demux18/1 -> Transform1/1(roll)
  Demux18/2 -> Transform1/2(pitch)
  Demux28/3 -> Transform2/6(MP_Z)
  Demux28/2 -> Transform2/5(MP_Y)
  Demux28/1 -> Transform2/4(MP_X)
  Demux27/1 -> Transform2/1(roll)
  Demux27/3 -> Transform2/3(yaw)
  Demux27/2 -> Transform2/2(pitch)
  Demux23/3 -> Transform6/6(MP_Z)
  Demux23/2 -> Transform6/5(MP_Y)
  Demux23/1 -> Transform6/4(MP_X)
  Demux25/3 -> Transform7/6(MP_Z)
  Demux25/2 -> Transform7/5(MP_Y)
  Demux25/1 -> Transform7/4(MP_X)
  Demux24/1 -> Transform7/1(roll)
  Demux24/3 -> Transform7/3(yaw)
  Demux24/2 -> Transform7/2(pitch)
  Transform3/3(MP_U4_Z) -> Mux12/3
  Transform2/3(MP_U3_Z) -> Mux11/3
  Transform1/3(MP_U2_Z) -> Mux10/3
  Transform/3(MP_U1_Z) -> Display3/1, Mux9/3
  Transform4/3(MP_L1_Z) -> Mux13/3
  Transform5/3(MP_L2_Z) -> Mux14/3
  Transform6/3(MP_L3_Z) -> Mux15/3
  Transform7/3(MP_L4_Z) -> Mux16/3
  Demux32/3 -> Transform3/6(MP_Z)
  Demux32/2 -> Transform3/5(MP_Y)
  Demux32/1 -> Transform3/4(MP_X)
  Demux29/3 -> Transform3/3(yaw)
  Demux29/2 -> Transform3/2(pitch)
  Demux29/1 -> Transform3/1(roll)
  Demux31/3 -> Transform/6(MP_Z)
  Demux33/1 -> Transform4/1(roll)
  Demux33/2 -> Transform4/2(pitch)
  Demux33/3 -> Transform4/3(yaw)
  Demux19/1 -> Transform4/4(MP_X)
  Demux19/2 -> Transform4/5(MP_Y)
  Demux19/3 -> Transform4/6(MP_Z)
  Demux20/1 -> Transform5/1(roll)
  Demux20/2 -> Transform5/2(pitch)
  Demux20/3 -> Transform5/3(yaw)
  Demux21/1 -> Transform5/4(MP_X)
  Demux21/2 -> Transform5/5(MP_Y)
  Demux21/3 -> Transform5/6(MP_Z)
  Demux22/1 -> Transform6/1(roll)
  Demux22/2 -> Transform6/2(pitch)
  Demux22/3 -> Transform6/3(yaw)

== system cable_driven_parallel_robot/Actuators-CableTension-MovingPlatform/2 Wheels Diffrential Mobile Robot/2 Wheels Diffrential Mobile Robot/Vel_Manager ==
  Demux : Demux  Outputs=3
  Demux1 : Demux  Outputs=8
  Terminator{,1..6} (7 alike) : Terminator
  Vx_min : Outport
  Vy_min : Outport  Port=2
  Vz_min : Outport  Port=3
  Reste : Outport  Port=4
  wires:
  [Vmin] -> Demux/1
  [isTension] -> Demux1/1
  Demux/1 -> Vx_min/1
  Demux/2 -> Vy_min/1
  Demux/3 -> Vz_min/1
  Demux1/5 -> Reste/1
  Demux1/1 -> Terminator/1
  Demux1/2 -> Terminator1/1
  Demux1/3 -> Terminator2/1
  Demux1/4 -> Terminator3/1
  Demux1/8 -> Terminator6/1
  Demux1/7 -> Terminator5/1
  Demux1/6 -> Terminator4/1

== system cable_driven_parallel_robot/Actuators-CableTension-MovingPlatform/2 Wheels Diffrential Mobile Robot/2 Wheels Diffrential Mobile Robot/wrap angle (Rad) ==
  angle_in : Inport
  Atan2 : Trigonometry  Operator=atan2
  Sin : Trigonometry
  cos : Trigonometry  Operator=cos
  angle_out : Outport
  wires:
  cos/1 -> Atan2/2
  Atan2/1 -> angle_out/1
  Sin/1 -> Atan2/1
  angle_in/1 -> Sin/1, cos/1

== system cable_driven_parallel_robot/Actuators-CableTension-MovingPlatform/2 Wheels Diffrential Mobile Robot1/2 Wheels Diffrential Mobile Robot/Vel_Manager ==
  Demux : Demux  Outputs=3
  Demux1 : Demux  Outputs=8
  Terminator{,1..6} (7 alike) : Terminator
  Vx_min : Outport
  Vy_min : Outport  Port=2
  Vz_min : Outport  Port=3
  Reste : Outport  Port=4
  wires:
  [Vmin] -> Demux/1
  [isTension] -> Demux1/1
  Demux/1 -> Vx_min/1
  Demux/2 -> Vy_min/1
  Demux/3 -> Vz_min/1
  Demux1/1 -> Terminator/1
  Demux1/2 -> Terminator1/1
  Demux1/3 -> Terminator2/1
  Demux1/4 -> Terminator3/1
  Demux1/8 -> Terminator6/1
  Demux1/7 -> Terminator5/1
  Demux1/6 -> Reste/1
  Demux1/5 -> Terminator4/1

== system cable_driven_parallel_robot/Actuators-CableTension-MovingPlatform/2 Wheels Diffrential Mobile Robot1/2 Wheels Diffrential Mobile Robot/wrap angle (Rad) ==
  angle_in : Inport
  Atan2 : Trigonometry  Operator=atan2
  Sin : Trigonometry
  cos : Trigonometry  Operator=cos
  angle_out : Outport
  wires:
  angle_in/1 -> cos/1, Sin/1
  Sin/1 -> Atan2/1
  Atan2/1 -> angle_out/1
  cos/1 -> Atan2/2

== system cable_driven_parallel_robot/Actuators-CableTension-MovingPlatform/2 Wheels Diffrential Mobile Robot2/2 Wheels Diffrential Mobile Robot/Vel_Manager ==
  Demux : Demux  Outputs=3
  Demux1 : Demux  Outputs=8
  Terminator{,1..6} (7 alike) : Terminator
  Vx_min : Outport
  Vy_min : Outport  Port=2
  Vz_min : Outport  Port=3
  Reste : Outport  Port=4
  wires:
  [Vmin] -> Demux/1
  [isTension] -> Demux1/1
  Demux/1 -> Vx_min/1
  Demux/2 -> Vy_min/1
  Demux/3 -> Vz_min/1
  Demux1/1 -> Terminator/1
  Demux1/2 -> Terminator1/1
  Demux1/3 -> Terminator2/1
  Demux1/4 -> Terminator3/1
  Demux1/8 -> Terminator6/1
  Demux1/7 -> Reste/1
  Demux1/6 -> Terminator4/1
  Demux1/5 -> Terminator5/1

== system cable_driven_parallel_robot/Actuators-CableTension-MovingPlatform/2 Wheels Diffrential Mobile Robot2/2 Wheels Diffrential Mobile Robot/wrap angle (Rad) ==
  angle_in : Inport
  Atan2 : Trigonometry  Operator=atan2
  Sin : Trigonometry
  cos : Trigonometry  Operator=cos
  angle_out : Outport
  wires:
  angle_in/1 -> cos/1, Sin/1
  Sin/1 -> Atan2/1
  Atan2/1 -> angle_out/1
  cos/1 -> Atan2/2

== system cable_driven_parallel_robot/Actuators-CableTension-MovingPlatform/2 Wheels Diffrential Mobile Robot3/2 Wheels Diffrential Mobile Robot/Vel_Manager ==
  Demux : Demux  Outputs=3
  Demux1 : Demux  Outputs=8
  Terminator{,1..6} (7 alike) : Terminator
  Vx_min : Outport
  Vy_min : Outport  Port=2
  Vz_min : Outport  Port=3
  Reste : Outport  Port=4
  wires:
  [Vmin] -> Demux/1
  [isTension] -> Demux1/1
  Demux/1 -> Vx_min/1
  Demux/2 -> Vy_min/1
  Demux/3 -> Vz_min/1
  Demux1/1 -> Terminator/1
  Demux1/2 -> Terminator1/1
  Demux1/3 -> Terminator2/1
  Demux1/4 -> Terminator3/1
  Demux1/5 -> Terminator5/1
  Demux1/8 -> Reste/1
  Demux1/6 -> Terminator4/1
  Demux1/7 -> Terminator6/1

== system cable_driven_parallel_robot/Actuators-CableTension-MovingPlatform/2 Wheels Diffrential Mobile Robot3/2 Wheels Diffrential Mobile Robot/wrap angle (Rad) ==
  angle_in : Inport
  Atan2 : Trigonometry  Operator=atan2
  Sin : Trigonometry
  cos : Trigonometry  Operator=cos
  angle_out : Outport
  wires:
  angle_in/1 -> cos/1, Sin/1
  Sin/1 -> Atan2/1
  Atan2/1 -> angle_out/1
  cos/1 -> Atan2/2

== system cable_driven_parallel_robot/Actuators-CableTension-MovingPlatform/Moving Platform/Moving Platform/Subsystem1 ==
  rest : Inport
  init : Inport  Port=2
  MATLAB Function : MATLAB Function  TreatAsAtomicUnit=on
  A_rest : Outport
  A_init : Outport  Port=2
  wires:
  rest/1 -> MATLAB Function/1(rest0)
  MATLAB Function/1(rest) -> A_rest/1
  init/1 -> MATLAB Function/2(init0)
  MATLAB Function/2(init) -> A_init/1

== system cable_driven_parallel_robot/Actuators-CableTension-MovingPlatform/Moving Platform/Moving Platform/Vel_Manager ==
  Demux : Demux  Outputs=3
  Demux1 : Demux  Outputs=8
  OR : Logic  Operator=OR  Inputs=8  IconShape=distinctive  AllPortsSameDT=off  OutDataTypeStr=boolean
  Vx_min : Outport
  Vy_min : Outport  Port=2
  Vz_min : Outport  Port=3
  Reste : Outport  Port=4
  wires:
  [Vmin] -> Demux/1
  [isTension] -> Demux1/1
  Demux/1 -> Vx_min/1
  Demux/2 -> Vy_min/1
  Demux/3 -> Vz_min/1
  Demux1/1 -> OR/1
  Demux1/2 -> OR/2
  Demux1/3 -> OR/3
  Demux1/4 -> OR/4
  Demux1/5 -> OR/5
  Demux1/6 -> OR/6
  Demux1/7 -> OR/7
  Demux1/8 -> OR/8
  OR/1 -> Reste/1

== system cable_driven_parallel_robot/Actuators-CableTension-MovingPlatform/Moving Platform/Moving Platform/wrap angle (Rad) ==
  angle_in : Inport
  Atan2 : Trigonometry  Operator=atan2
  Sin : Trigonometry
  cos : Trigonometry  Operator=cos
  angle_out : Outport
  wires:
  cos/1 -> Atan2/2
  Atan2/1 -> angle_out/1
  Sin/1 -> Atan2/1
  angle_in/1 -> Sin/1, cos/1

== system cable_driven_parallel_robot/Actuators-CableTension-MovingPlatform/Moving Platform/Moving Platform/wrap angle (Rad)1 ==
  angle_in : Inport
  Atan2 : Trigonometry  Operator=atan2
  Sin : Trigonometry
  cos : Trigonometry  Operator=cos
  angle_out : Outport
  wires:
  angle_in/1 -> cos/1, Sin/1
  Sin/1 -> Atan2/1
  Atan2/1 -> angle_out/1
  cos/1 -> Atan2/2

== system cable_driven_parallel_robot/Actuators-CableTension-MovingPlatform/Moving Platform/Moving Platform/wrap angle (Rad)2 ==
  angle_in : Inport
  Atan2 : Trigonometry  Operator=atan2
  Sin : Trigonometry
  cos : Trigonometry  Operator=cos
  angle_out : Outport
  wires:
  cos/1 -> Atan2/2
  Atan2/1 -> angle_out/1
  Sin/1 -> Atan2/1
  angle_in/1 -> Sin/1, cos/1

== system cable_driven_parallel_robot/Actuators-CableTension-MovingPlatform/QuadRotor/Subsystem/Subsystem ==
  rest : Inport
  init : Inport  Port=2
  MATLAB Function : MATLAB Function  TreatAsAtomicUnit=on
  A_rest : Outport
  A_init : Outport  Port=2
  wires:
  rest/1 -> MATLAB Function/1(rest0)
  MATLAB Function/1(rest) -> A_rest/1
  init/1 -> MATLAB Function/2(init0)
  MATLAB Function/2(init) -> A_init/1

== system cable_driven_parallel_robot/Actuators-CableTension-MovingPlatform/QuadRotor/Subsystem/Subsystem1 ==
  rest : Inport
  init : Inport  Port=2
  MATLAB Function : MATLAB Function  TreatAsAtomicUnit=on
  A_rest : Outport
  A_init : Outport  Port=2
  wires:
  rest/1 -> MATLAB Function/1(rest0)
  MATLAB Function/1(rest) -> A_rest/1
  init/1 -> MATLAB Function/2(init0)
  MATLAB Function/2(init) -> A_init/1

== system cable_driven_parallel_robot/Actuators-CableTension-MovingPlatform/QuadRotor/Subsystem/Vel_Manager ==
  Demux : Demux  Outputs=3
  Demux1 : Demux  Outputs=8
  Terminator{,1..6} (7 alike) : Terminator
  Vx_min : Outport
  Vy_min : Outport  Port=2
  Vz_min : Outport  Port=3
  Reste : Outport  Port=4
  wires:
  Demux1/7 -> Terminator5/1
  Demux1/3 -> Terminator1/1
  [Vmin] -> Demux/1
  Demux1/8 -> Terminator6/1
  [isTension] -> Demux1/1
  Demux1/6 -> Terminator4/1
  Demux1/2 -> Terminator/1
  Demux1/5 -> Terminator3/1
  Demux1/4 -> Terminator2/1
  Demux/1 -> Vx_min/1
  Demux/2 -> Vy_min/1
  Demux/3 -> Vz_min/1
  Demux1/1 -> Reste/1
